simulink model "EV6_LUT_FourWheel_EV6Battery77p4kWh_PowerCorrected"  (R2024a)
settings: Solver=ode4  StartTime=0  StopTime=60  FixedStep=0.001  RelTol=1e-3
PreLoadFcn:
  | VSS_BICYCLE=Simulink.Variant('Dual=0');
  | VSS_DUAL=Simulink.Variant('Dual=1');
  | Dual=1;
  | load('DriveCycle2.mat')
PostLoadFcn:
  | if any(exist('dsrtsu_mdlpostloadfcn', 'file') ~= 0), dsrtsu_mdlpostloadfcn('Execute', bdroot); end
InitFcn:
  | , if any(exist('rtifpga_mdlclblib', 'file') ~= 0), rtifpga_mdlclblib('Init', bdroot); end,
  | , if any(exist('dsmpb_private', 'file') ~= 0), dsmpb_private('dsmpb_mdlclblib', 'Init', bdroot); end,
  | load('DriveCycle2.mat')
model workspace (MAT data in the model file):
  DiffRatio = 10.65
  EV6_2023_BattBranchCapacity_Ah = 55.5236728838
  EV6_2023_BattEnergy_kWh = 77.4
  EV6_2023_BattNominalVoltage_V = 697
  EV6_2023_BattNumCellsParallel = 2
  EV6_2023_BattNumCellsSeries = 192
  EV6_2023_BattOpenVoltCapBpts = [0 0.1 0.2 0.3 0.4 0.5 0.6 0.7 0.8 0.9 1]
  EV6_2023_BattOpenVoltTbl = [2.96762142548 3.40364281191 3.47417488548 3.54470541822 3.61523441014 3.68576186124 3.75628777151 3.82681214095 3.94527005036 4.07101207308 4.2120755254]
  EV6_2023_BattPackCapacity_Ah = 111.047345768
  EV6_2023_BattResistSocBpts = [0 0.2 0.4 0.6 0.8 1]
  EV6_2023_BattResistTbl = [0.0163620057716 0.0118174152018 0.00807187352333 0.00375663957972 0.00266904525531 0.00103635901355 0.0019014404175 0.0172368903217 0.0121226074867 0.00758541551769 0.00474065349228 0.00337561163613 ... (42 elements, 7x6)]
  EV6_2023_BattResistTempBpts = [243.1 253.1 263.1 273.1 283.1 298.1 313.1]
  EV6_2023_InitialPackOCV_V = 726.471714233
  EV6_2023_InitialSOC = 0.638878863672
  EV6_BattCellCapacity_Ah = 60.3
  EV6_BattInitialSOC = 0.638878863672
  EV6_BattOCV_Cell_V = [2.96762142548 3.40364281191 3.47417488548 3.54470541822 3.61523441014 3.68576186124 3.75628777151 3.82681214095 3.94527005036 4.07101207308 4.2120755254]
  EV6_BattOCV_SOC = [0 0.1 0.2 0.3 0.4 0.5 0.6 0.7 0.8 0.9 1]
  EV6_BattPackCapacity_Ah = 120.6
  EV6_BattParallelCells = 2
  EV6_BattResistanceSOC = [0 0.2 0.4 0.6 0.8 1]
  EV6_BattResistanceTable_Ohm = [0.0163620057716 0.0118174152018 0.00807187352333 0.00375663957972 0.00266904525531 0.00103635901355 0.0019014404175 0.0172368903217 0.0121226074867 0.00758541551769 0.00474065349228 0.00337561163613 ... (42 elements, 7x6)]
  EV6_BattResistanceTemp_K = [243.1 253.1 263.1 273.1 283.1 298.1 313.1]
  EV6_BattSeriesCells = 192
  EV6_FinalDriveRatio = 10.65
  EV6_TargetPackResistance_Ohm = 0.132763804608
  Gas = 0.383333333333
undefined symbols (not defined in the file): accel_bp_mps2, AccelCmd, ActTqLF_Nm_, ActTqLR_Nm_, ActTqRF_Nm_, ActTqRR_Nm_, BattChargeLimitMaxPwr, BattChargeLimitSocBpts, BattChargeLimitTbl, BattDischargeLimitSocBpts, BattDischargeLimitTbl, BattDischargeMaxPwr, BrakeMaxPrs, BrakeMaxTrq, ChassisDistCg2FrontAxle, ChassisDistCg2RearAxle, ChassisVehMass, CltchCmd, CoastDown, DecelCmd, DiscIntNeverNeededParam, EnvGravCnst, EnvPrs, EnvTemp, EV6_RegenTorqueGain, EV6_TractionTorqueGain, front_share_regen_3d, front_share_traction_3d, FuelSpecificGrav, GearCmd, h, InitStates, lgSw, limitedMCT, MCT, MtrEffSpdBpts, MtrEffTbl, MtrEffTrqBpts, MtrPwrMax, MtrTrqMax, out_1, pMCT, RealSimPara, Ref_speed, Ref_time, regen_torque_bp_Nm, speed_bp_kph, SteeringCmd, SupvsryCtrlRegenBrkCutOffTbl, SupvsryCtrlRegenSpdBpts, TestScnrioCycleNum, traction_torque_bp_Nm, US06, VEH
libraries: VSIGenLib x65, simulink x54, etargetslib x38, dsmpblib x24, vehdynlibtire x12, autolibshared x11, vehdynlibsuspension x7, vehdynlibtirecommon x7, autolibpowerinfoutils x6, autolibutils x5, autolibsharedcoupling x4, autolibmappedmotor x4
(part 2 of 19)

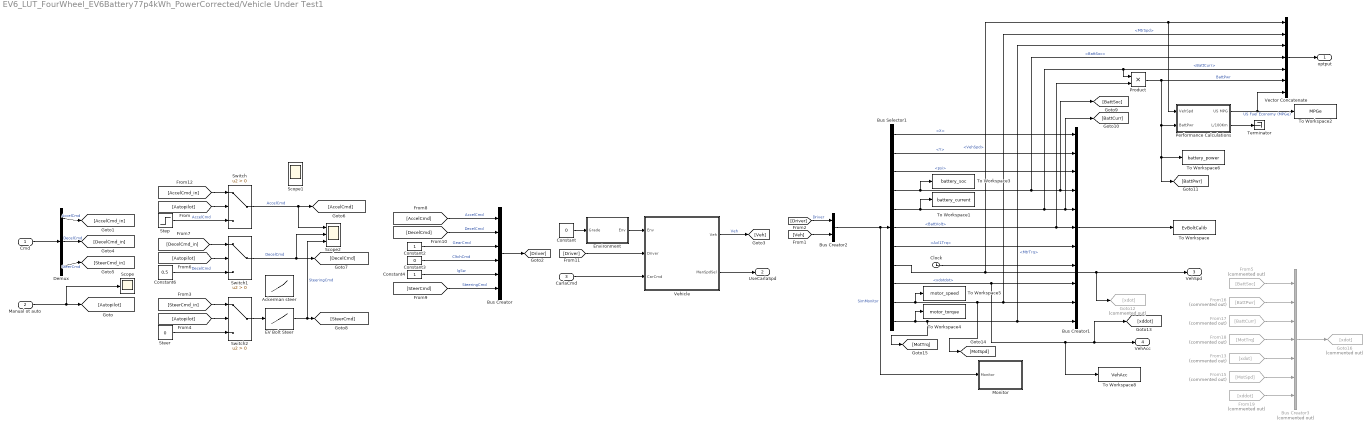
== system EV6_LUT_FourWheel_EV6Battery77p4kWh_PowerCorrected/Vehicle Under Test1 ==
  Cmd : Inport
  Manual ot auto : Inport  Port=2
  CarlaCmd : Inport  Port=3
  Ackerman steer : Lookup_n-D  NumberOfTableDimensions=1  BreakpointsForDimension1="[-0.446316297916244\t-0.442150786830951\t-0.437977161945005\t-0.433795286969319\t-0.429605025209166\t-0.425406239561593\t-0.421198792513030\t-0.416982546137136\t-0.412757362092861\t-0.408523101622746\t-0.404279625551461\t-0.400026794284603\t-0.395764467807732\t-0.391492505685692\t-0.387210767062193\t-0.382919110659678\t-0.378617394779480\t-0.374305477302279\t-0.369983215688866\t-0.365650466981227\t-0.361307087803951\t-0.356952934365975\t-0.352587862462675\t-0.348211727478321\t-0.343824384388886\t-0.339425687765245\t-0.335015491776758\t-0.330593650195247\t-0.326160016399396\t-0.321714443379563\t-0.317256783743034\t-0.312786889719717\t-0.308304613168298\t-0.303809805582871\t-0.299302318100048\t-0.294782001506567\t-0.290248706247410\t-0.285702282434450\t-0.281142579855627\t-0.276569447984685\t-0.271982735991464\t-0.267382292752788\t-0.262767966863931\t-0.258139606650706\t-0.253497060182174\t-0.248840175283994\t-0.244168799552432\t-0.239482780369037\t-0.234781964916014\t-0.230066200192295\t-0.225335333030331\t-0.220589210113630\t-0.215827677995039\t-0.211050583115807\t-0.206257771825433\t-0.201449090402323\t-0.196624385075265\t-0.191783502045761\t-0.186926287511198\t-0.182052587688919\t-0.177162248841170\t-0.172255117300976\t-0.167331039498945\t-0.162389861991014\t-0.157431431487183\t-0.152455594881217\t-0.147462199281363\t-0.142451092042095\t-0.137422120796894\t-0.132375133492088\t-0.127309978421782\t-0.122226504263869\t-0.117124560117169\t-0.112003995539695\t-0.106864660588066\t-0.101706405858090\t-0.0965290825265349\t-0.0913325423940914\t-0.0861166379295599\t-0.0808812223152671\t-0.0756261494937309\t-0.0703512742155897\t-0.0650564520888085\t-0.0597415396291770\t-0.0544063943121130\t-0.0490508746257825\t-0.0436748401255510\t-0.0382781514897739\t-0.0328606705769398\t-0.0274222604841732\t-0.0219627856071077\t-0.0164821117011354\t-0.0109801059440403\t-0.00545663700002112\t0\t0.00547767577609933\t0.0110656090794470\t0.0166755107772618\t0.0223075038233658\t0.0279617092740365\t0.0336382462142580\t0.0393372316825870\t0.0450587805946413\t0.0508030056652199\t0.0565700173290652\t0.0623599236602815\t0.0681728302904245\t0.0740088403252790\t0.0798680542603446\t0.0857505698950509\t0.0916564822457268\t0.0975858834573503\t0.103538862714108\t0.109515506148794\t0.115515896751090\t0.121540114274751\t0.127588235143750\t0.133660332357415\t0.139756475394610\t0.145876730117007\t0.152021158671496\t0.158189819391799\t0.164382766699339\t0.170600051003425\t0.176841718600822\t0.183107811574771\t0.189398367693541\t0.195713420308563\t0.202052998252265\t0.208417125735647\t0.214805822245717\t0.221219102442855\t0.227656976058216\t0.234119447791246\t0.240606517207442\t0.247118178636427\t0.253654421070478\t0.260215228063589\t0.266800577631217\t0.273410442150791\t0.280044788263140\t0.286703576774936\t0.293386762562311\t0.300094294475738\t0.306826115246357\t0.313582161393837\t0.320362363135953\t0.327166644299990\t0.333994922236136\t0.340847107733006\t0.347723104935443\t0.354622811264752\t0.361546117341510\t0.368492906911125\t0.375463056772267\t0.382456436708368\t0.389472909422305\t0.396512330474460\t0.403574548224288\t0.410659403775562\t0.417766730925451\t0.424896356117582\t0.432048098399246\t0.439221769382891\t0.446417173212069\t0.453634106531970\t0.460872358464695\t0.468131710589418\t0.475411936927561\t0.482712803933137\t0.490034070488372\t0.497375487904758\t0.504736799929627\t0.512117742758400\t0.519518045052588\t0.526937427963674\t0.534375605162959\t0.541832282877473\t0.549307159932028\t0.556799927797496\t0.564310270645373\t0.571837865408689\t0.579382381849329\t0.586943482631776\t0.594520823403350\t0.602114052880920\t0.609722812944144\t0.617346738735206\t0.624985458765058]"  Table="[-9.40000000000000\t-9.30000000000000\t-9.20000000000000\t-9.10000000000000\t-9\t-8.90000000000000\t-8.80000000000000\t-8.70000000000000\t-8.60000000000000\t-8.50000000000000\t-8.40000000000000\t-8.30000000000000\t-8.20000000000000\t-8.10000000000000\t-8\t-7.90000000000000\t-7.80000000000000\t-7.70000000000000\t-7.60000000000000\t-7.50000000000000\t-7.40000000000000\t-7.30000000000000\t-7.20000000000000\t-7.10000000000000\t-7\t-6.90000000000000\t-6.80000000000000\t-6.70000000000000\t-6.60000000000000\t-6.50000000000000\t-6.40000000000000\t-6.30000000000000\t-6.20000000000000\t-6.10000000000000\t-6\t-5.90000000000000\t-5.80000000000000\t-5.70000000000000\t-5.60000000000000\t-5.50000000000000\t-5.40000000000000\t-5.30000000000000\t-5.20000000000000\t-5.10000000000000\t-5\t-4.90000000000000\t-4.80000000000000\t-4.70000000000000\t-4.60000000000000\t-4.50000000000000\t-4.40000000000000\t-4.30000000000000\t-4.20000000000000\t-4.10000000000000\t-4\t-3.90000000000000\t-3.80000000000000\t-3.70000000000000\t-3.60000000000000\t-3.50000000000000\t-3.40000000000000\t-3.30000000000000\t-3.20000000000000\t-3.10000000000000\t-3\t-2.90000000000000\t-2.80000000000000\t-2.70000000000000\t-2.60000000000000\t-2.50000000000000\t-2.40000000000000\t-2.30000000000000\t-2.20000000000000\t-2.10000000000000\t-2\t-1.90000000000000\t-1.80000000000000\t-1.70000000000000\t-1.60000000000000\t-1.50000000000000\t-1.40000000000000\t-1.30000000000000\t-1.20000000000000\t-1.10000000000000\t-1\t-0.900000000000000\t-0.800000000000000\t-0.700000000000000\t-0.600000000000000\t-0.500000000000000\t-0.400000000000000\t-0.300000000000000\t-0.200000000000000\t-0.100000000000000\t0\t0.100000000000000\t0.200000000000000\t0.300000000000000\t0.400000000000000\t0.500000000000000\t0.600000000000000\t0.700000000000000\t0.800000000000000\t0.900000000000000\t1\t1.10000000000000\t1.20000000000000\t1.30000000000000\t1.40000000000000\t1.50000000000000\t1.60000000000000\t1.70000000000000\t1.80000000000000\t1.90000000000000\t2\t2.10000000000000\t2.20000000000000\t2.30000000000000\t2.40000000000000\t2.50000000000000\t2.60000000000000\t2.70000000000000\t2.80000000000000\t2.90000000000000\t3\t3.10000000000000\t3.20000000000000\t3.30000000000000\t3.40000000000000\t3.50000000000000\t3.60000000000000\t3.70000000000000\t3.80000000000000\t3.90000000000000\t4\t4.10000000000000\t4.20000000000000\t4.30000000000000\t4.40000000000000\t4.50000000000000\t4.60000000000000\t4.70000000000000\t4.80000000000000\t4.90000000000000\t5\t5.10000000000000\t5.20000000000000\t5.30000000000000\t5.40000000000000\t5.50000000000000\t5.60000000000000\t5.70000000000000\t5.80000000000000\t5.90000000000000\t6\t6.10000000000000\t6.20000000000000\t6.30000000000000\t6.40000000000000\t6.50000000000000\t6.60000000000000\t6.70000000000000\t6.80000000000000\t6.90000000000000\t7\t7.10000000000000\t7.20000000000000\t7.30000000000000\t7.40000000000000\t7.50000000000000\t7.60000000000000\t7.70000000000000\t7.80000000000000\t7.90000000000000\t8\t8.10000000000000\t8.20000000000000\t8.30000000000000\t8.40000000000000\t8.50000000000000\t8.60000000000000\t8.70000000000000\t8.80000000000000\t8.90000000000000\t9\t9.10000000000000\t9.20000000000000\t9.30000000000000\t9.40000000000000]"  InternalRulePriority=Speed  RndMeth=Simplest
  Bus Creator : BusCreator  Inputs=AccelCmd,DecelCmd,GearCmd,CltchCmd,lgSw,SteeringCmd
  Bus Creator1 : BusCreator  Inputs=11
  Bus Creator2 : BusCreator  Inputs=2
  Bus Creator3 : BusCreator  Commented=on  Inputs=7
  Bus Selector1 : BusSelector  OutputSignals=Veh.Chassis.X,Veh.Chassis.Y,Veh.Chassis.psi,Veh.Batt.BattSoc,Veh.Batt.BattCurr,Veh.Batt.BattVolt,Veh.Diff.Axl1.Axl1Trq,Veh.Chassis.VehSpd,Veh.Chassis.xdotdot,Veh.Mtr.MtrSpd,Veh.Mtr.MtrTrq
  Clock : Clock
  Constant : Constant  Value=0
  Constant2 : Constant
  Constant3 : Constant  Value=0
  Constant4 : Constant
  Constant6 : Constant  Value=0.5  SampleTime=-1
  Demux : Demux  Outputs=3
  EV Bolt Steer : Lookup_n-D  NumberOfTableDimensions=1  BreakpointsForDimension1="[-0.541571931581492\t-0.535619550629112\t-0.529667169676731\t-0.523714788724350\t-0.517762407771969\t-0.511810026819588\t-0.505857645867207\t-0.499905264914826\t-0.493952883962445\t-0.488000503010064\t-0.482048122057683\t-0.476095741105302\t-0.470143360152921\t-0.464190979200541\t-0.458238598248160\t-0.452286217295779\t-0.446333836343398\t-0.440381455391017\t-0.434429074438636\t-0.428476693486255\t-0.422524312533874\t-0.416571931581493\t-0.410619550629112\t-0.404667169676731\t-0.398714788724350\t-0.392762407771969\t-0.386810026819588\t-0.380857645867207\t-0.374905264914826\t-0.368952883962445\t-0.363000503010064\t-0.357048122057683\t-0.351095741105302\t-0.345143360152921\t-0.339190979200541\t-0.333238598248160\t-0.327286217295779\t-0.321333836343398\t-0.315381455391017\t-0.309429074438636\t-0.303476693486255\t-0.297524312533874\t-0.291571931581493\t-0.285619550629112\t-0.279667169676731\t-0.273714788724350\t-0.267762407771969\t-0.261810026819588\t-0.255857645867207\t-0.249905264914826\t-0.243952883962445\t-0.238000503010065\t-0.232048122057684\t-0.226095741105303\t-0.220143360152922\t-0.214190979200541\t-0.208238598248160\t-0.202286217295779\t-0.196333836343398\t-0.190381455391017\t-0.184429074438636\t-0.178476693486255\t-0.172524312533874\t-0.166571931581493\t-0.160619550629112\t-0.154667169676731\t-0.148714788724350\t-0.142762407771969\t-0.136810026819588\t-0.130857645867207\t-0.124905264914826\t-0.118952883962445\t-0.113000503010064\t-0.107048122057683\t-0.101095741105303\t-0.0951433601529216\t-0.0891909792005406\t-0.0832385982481596\t-0.0772862172957787\t-0.0713338363433977\t-0.0653814553910168\t-0.0594290744386358\t-0.0534766934862548\t-0.0475243125338739\t-0.0415719315814929\t-0.0356195506291120\t-0.0296671696767310\t-0.0237147887243500\t-0.0177624077719691\t-0.0118100268195881\t-0.00585764586720720\t0\t0.00585764586720720\t0.0118100268195881\t0.0177624077719691\t0.0237147887243500\t0.0296671696767310\t0.0356195506291120\t0.0415719315814929\t0.0475243125338739\t0.0534766934862548\t0.0594290744386358\t0.0653814553910168\t0.0713338363433977\t0.0772862172957787\t0.0832385982481596\t0.0891909792005406\t0.0951433601529216\t0.101095741105303\t0.107048122057683\t0.113000503010064\t0.118952883962445\t0.124905264914826\t0.130857645867207\t0.136810026819588\t0.142762407771969\t0.148714788724350\t0.154667169676731\t0.160619550629112\t0.166571931581493\t0.172524312533874\t0.178476693486255\t0.184429074438636\t0.190381455391017\t0.196333836343398\t0.202286217295779\t0.208238598248160\t0.214190979200541\t0.220143360152922\t0.226095741105303\t0.232048122057684\t0.238000503010065\t0.243952883962445\t0.249905264914826\t0.255857645867207\t0.261810026819588\t0.267762407771969\t0.273714788724350\t0.279667169676731\t0.285619550629112\t0.291571931581493\t0.297524312533874\t0.303476693486255\t0.309429074438636\t0.315381455391017\t0.321333836343398\t0.327286217295779\t0.333238598248160\t0.339190979200541\t0.345143360152921\t0.351095741105302\t0.357048122057683\t0.363000503010064\t0.368952883962445\t0.374905264914826\t0.380857645867207\t0.386810026819588\t0.392762407771969\t0.398714788724350\t0.404667169676731\t0.410619550629112\t0.416571931581493\t0.422524312533874\t0.428476693486255\t0.434429074438636\t0.440381455391017\t0.446333836343398\t0.452286217295779\t0.458238598248160\t0.464190979200541\t0.470143360152921\t0.476095741105302\t0.482048122057683\t0.488000503010064\t0.493952883962445\t0.499905264914826\t0.505857645867207\t0.511810026819588\t0.517762407771969\t0.523714788724350\t0.529667169676731\t0.535619550629112\t0.541571931581492]"  Table="[-9.10000000000000\t-9\t-8.90000000000000\t-8.80000000000000\t-8.70000000000000\t-8.60000000000000\t-8.50000000000000\t-8.40000000000000\t-8.30000000000000\t-8.20000000000000\t-8.10000000000000\t-8\t-7.90000000000000\t-7.80000000000000\t-7.70000000000000\t-7.60000000000000\t-7.50000000000000\t-7.40000000000000\t-7.30000000000000\t-7.20000000000000\t-7.10000000000000\t-7\t-6.90000000000000\t-6.80000000000000\t-6.70000000000000\t-6.60000000000000\t-6.50000000000000\t-6.40000000000000\t-6.30000000000000\t-6.20000000000000\t-6.10000000000000\t-6\t-5.90000000000000\t-5.80000000000000\t-5.70000000000000\t-5.60000000000000\t-5.50000000000000\t-5.40000000000000\t-5.30000000000000\t-5.20000000000000\t-5.10000000000000\t-5\t-4.90000000000000\t-4.80000000000000\t-4.70000000000000\t-4.60000000000000\t-4.50000000000000\t-4.40000000000000\t-4.30000000000000\t-4.20000000000000\t-4.10000000000000\t-4\t-3.90000000000000\t-3.80000000000000\t-3.70000000000000\t-3.60000000000000\t-3.50000000000000\t-3.40000000000000\t-3.30000000000000\t-3.20000000000000\t-3.10000000000000\t-3\t-2.90000000000000\t-2.80000000000000\t-2.70000000000000\t-2.60000000000000\t-2.50000000000000\t-2.40000000000000\t-2.30000000000000\t-2.20000000000000\t-2.10000000000000\t-2\t-1.90000000000000\t-1.80000000000000\t-1.70000000000000\t-1.60000000000000\t-1.50000000000000\t-1.40000000000000\t-1.30000000000000\t-1.20000000000000\t-1.10000000000000\t-1\t-0.900000000000000\t-0.800000000000000\t-0.700000000000000\t-0.600000000000000\t-0.500000000000000\t-0.400000000000000\t-0.300000000000000\t-0.200000000000000\t-0.100000000000000\t0\t0.100000000000000\t0.200000000000000\t0.300000000000000\t0.400000000000000\t0.500000000000000\t0.600000000000000\t0.700000000000000\t0.800000000000000\t0.900000000000000\t1\t1.10000000000000\t1.20000000000000\t1.30000000000000\t1.40000000000000\t1.50000000000000\t1.60000000000000\t1.70000000000000\t1.80000000000000\t1.90000000000000\t2\t2.10000000000000\t2.20000000000000\t2.30000000000000\t2.40000000000000\t2.50000000000000\t2.60000000000000\t2.70000000000000\t2.80000000000000\t2.90000000000000\t3\t3.10000000000000\t3.20000000000000\t3.30000000000000\t3.40000000000000\t3.50000000000000\t3.60000000000000\t3.70000000000000\t3.80000000000000\t3.90000000000000\t4\t4.10000000000000\t4.20000000000000\t4.30000000000000\t4.40000000000000\t4.50000000000000\t4.60000000000000\t4.70000000000000\t4.80000000000000\t4.90000000000000\t5\t5.10000000000000\t5.20000000000000\t5.30000000000000\t5.40000000000000\t5.50000000000000\t5.60000000000000\t5.70000000000000\t5.80000000000000\t5.90000000000000\t6\t6.10000000000000\t6.20000000000000\t6.30000000000000\t6.40000000000000\t6.50000000000000\t6.60000000000000\t6.70000000000000\t6.80000000000000\t6.90000000000000\t7\t7.10000000000000\t7.20000000000000\t7.30000000000000\t7.40000000000000\t7.50000000000000\t7.60000000000000\t7.70000000000000\t7.80000000000000\t7.90000000000000\t8\t8.10000000000000\t8.20000000000000\t8.30000000000000\t8.40000000000000\t8.50000000000000\t8.60000000000000\t8.70000000000000\t8.80000000000000\t8.90000000000000\t9\t9.10000000000000]"  InternalRulePriority=Speed  RndMeth=Simplest
  Environment : Subsystem
  From13 : From  Commented=on  GotoTag=xdot
  From15 : From  Commented=on  GotoTag=MotSpd
  From16 : From  Commented=on  GotoTag=BattPwr
  From17 : From  Commented=on  GotoTag=BattCurr
  From18 : From  Commented=on  GotoTag=MotTrq
  From19 : From  Commented=on  GotoTag=xddot
  From5 : From  Commented=on  GotoTag=BattSoc
  Goto12 : Goto  Commented=on  GotoTag=xdot
  Goto16 : Goto  Commented=on  GotoTag=xdot
  Monitor : Subsystem
  Performance Calculations : Subsystem
  Product : Product
  Scope : Scope
  Scope1 : Scope  NumInputPorts=3
  Scope2 : Scope  NumInputPorts=3
  Steer : Constant  Value=0
  Step : Step  Time=5  After=0
  Switch : Switch  Criteria=u2 > Threshold  SaturateOnIntegerOverflow=off  InputSameDT=off
  Switch1 : Switch  Criteria=u2 > Threshold  SaturateOnIntegerOverflow=off  InputSameDT=off
  Switch2 : Switch  Criteria=u2 > Threshold  SaturateOnIntegerOverflow=off  InputSameDT=off
  Terminator : Terminator
  To Workspace : ToWorkspace  VariableName=EvBoltCalib  SaveFormat=Structure With Time  SampleTime=-1
  To Workspace1 : ToWorkspace  VariableName=battery_current  SaveFormat=Timeseries  SampleTime=0.1
  To Workspace2 : ToWorkspace  VariableName=MPGe  SaveFormat=Timeseries  SampleTime=0.1
  To Workspace3 : ToWorkspace  VariableName=battery_soc  SaveFormat=Timeseries  SampleTime=0.1
  To Workspace4 : ToWorkspace  VariableName=motor_torque  SaveFormat=Timeseries  SampleTime=0.1
  To Workspace5 : ToWorkspace  VariableName=motor_speed  SaveFormat=Timeseries  SampleTime=0.1
  To Workspace6 : ToWorkspace  VariableName=battery_power  SaveFormat=Timeseries  SampleTime=0.1
  To Workspace8 : ToWorkspace  VariableName=VehAcc  SaveFormat=Timeseries  SampleTime=0.1
  Vector Concatenate : Concatenate  NumInputs=7
  Vehicle : Subsystem
  optput : Outport
  UseCarlaSpd : Outport  Port=2
  VehSpd : Outport  Port=3
  VehAcc : Outport  Port=4
  wires:
  Performance Calculations/2(L/100Km) -> Terminator/1
  Performance Calculations/1(US MPG) -> Vector Concatenate/7, To Workspace2/1  "US Fuel Economy (MPGe)"
  Product/1 -> Vector Concatenate/6, Performance Calculations/2(BattPwr), [BattPwr], To Workspace6/1  "BattPwr"
  Bus Selector1/11 -> [MotTrq], Vector Concatenate/3, Bus Creator1/11, To Workspace4/1  "<MtrTrq>"
  Bus Selector1/10 -> [MotSpd], Vector Concatenate/2, Bus Creator1/10, To Workspace5/1  "<MtrSpd>"
  [Driver] -> Vehicle/2(Driver)
  [DecelCmd] -> Bus Creator/2  "DecelCmd"
  EV Bolt Steer/1 -> [SteerCmd], Scope2/3  "SteeringCmd"
  [AccelCmd] -> Bus Creator/1  "AccelCmd"
  [DecelCmd_in] -> Switch1/1
  [Autopilot] -> Switch1/2
  [SteerCmd_in] -> Switch2/1
  [Autopilot] -> Switch2/2
  [AccelCmd_in] -> Switch/1
  Bus Selector1/9 -> To Workspace8/1, [xddot], VehAcc/1, Bus Creator1/9  "<xdotdot>"
  [Veh] -> Bus Creator2/2
  Vehicle/2(ManSpdSel) -> UseCarlaSpd/1
  CarlaCmd/1 -> Vehicle/3(CarCmd)
  Demux/3 -> [SteerCmd_in]  "SteerCmd"
  Steer/1 -> Switch2/3
  Demux/2 -> [DecelCmd_in]  "DecelCmd"
  Constant6/1 -> Switch1/3  "DecelCmd"
  Demux/1 -> [AccelCmd_in]  "AccelCmd"
  Step/1 -> Switch/3  "AccelCmd"
  [Autopilot] -> Switch/2
  Manual ot auto/1 -> [Autopilot], Scope/1
  Switch1/1 -> [DecelCmd], Scope2/2  "DecelCmd"
  Switch/1 -> [AccelCmd], Scope2/1  "AccelCmd"
  Switch2/1 -> EV Bolt Steer/1
  [SteerCmd] -> Bus Creator/6  "SteeringCmd"
  Bus Selector1/8 -> Vector Concatenate/1, Performance Calculations/1(VehSpd), Goto12/1, VehSpd/1  "<VehSpd>"
  Bus Selector1/7 -> Bus Creator1/7  "<Axl1Trq>"
  Bus Selector1/6 -> Bus Creator1/6, Product/2  "<BattVolt>"
  Bus Selector1/5 -> [BattCurr], Bus Creator1/5, Vector Concatenate/5, Product/1, To Workspace1/1  "<BattCurr>"
  Bus Selector1/4 -> Vector Concatenate/4, [BattSoc], Bus Creator1/4, To Workspace3/1  "<BattSoc>"
  Bus Selector1/3 -> Bus Creator1/3  "<psi>"
  Bus Selector1/2 -> Bus Creator1/2  "<Y>"
  Bus Selector1/1 -> Bus Creator1/1  "<X>"
  Clock/1 -> Bus Creator1/8
  Vector Concatenate/1 -> optput/1
  Constant2/1 -> Bus Creator/3  "GearCmd"
  Bus Creator1/1 -> To Workspace/1
  Constant4/1 -> Bus Creator/5  "lgSw"
  Constant/1 -> Environment/1(Grade)
  Environment/1(Env) -> Vehicle/1(Env)
  Vehicle/1(Veh) -> [Veh]  "Veh"
  Bus Creator/1 -> [Driver]
  Cmd/1 -> Demux/1
  Constant3/1 -> Bus Creator/4  "CltchCmd"
  [Driver] -> Bus Creator2/1  "Driver"
  Bus Creator2/1 -> Bus Selector1/1, Monitor/1(Monitor)  "SimMonitor"
  From5/1 -> Bus Creator3/1
  From16/1 -> Bus Creator3/2
  From17/1 -> Bus Creator3/3
  From18/1 -> Bus Creator3/4
  From13/1 -> Bus Creator3/5
  From15/1 -> Bus Creator3/6
  From19/1 -> Bus Creator3/7
  Bus Creator3/1 -> Goto16/1

== system EV6_LUT_FourWheel_EV6Battery77p4kWh_PowerCorrected/RealSim1/FromRealSim ==
  note: RealSimDepack
      | INPUTS
      | 0: uint8 ByteData array, this is message received from TrafficLayer
      | 1: nByte received
      |
      | The OUTPUTS can be customized based on the needs. Check SourceCode of this block for details.
  note: RealSimSocket
      | PARAMETERS:
      | 0: ip address of the RealSim TrafficLayer
      | 1: port to RealSim TrafficLayer
      | 2: enable log or not, disable for performance
      | INPUT:
      | 0: simulation time
      | 1: dt, frequency to receive and send to Traffic Simulator, has to be 0.1 for now, DO NOT change
      | 2: enable connection, 1: enable, 0: close. NOT currently used.
      | 3: ByteData to send
      | 4: nMsgSize
      |
      | OUTPUT:
      | 0: uint8 ByteData array
      | 1: nByte received
      | 2: connection flag, 1: connected to TrafficSimulator, 0: not connected
  tSimu : Inport
  dt : Inport  Port=2
  enableConnection : Inport  Port=3
  byteDataOut : Inport  Port=4
  nMsgSizeOut : Inport  Port=5
  Data Type Conversion1 : DataTypeConversion  OutDataTypeStr=uint8  SaturateOnIntegerOverflow=off  RndMeth=Floor
  Data Type Conversion2 : DataTypeConversion  OutDataTypeStr=boolean  SaturateOnIntegerOverflow=off  RndMeth=Floor
  Data Type Conversion3 : DataTypeConversion  OutDataTypeStr=double  SaturateOnIntegerOverflow=off  RndMeth=Floor
  Display8 : Display
  MATLAB System : MATLABSystem  System=RealSimDepack  OutputBusName=VehDataBus  VehicleMessageFieldDefInputVec=VehicleMessageFieldDefInputVec  SimulateUsing=Interpreted execution
      mask Type: RealSimDepack
      mask Display:
      | disp('RealSimDepack');
      | port_label('input',1,'ByteData');
      | port_label('input',2,'nByte');
      | port_label('input',3,'connectionState');
      | port_label('output',1,'simState');
      | port_label('output',2,'t');
      | port_label('output',3,'nVeh');
      | port_label('output',4,'VehDataBus');
      | port_label('output',5,'isVehicleInNetwork');
  S-Function : S-Function  FunctionName=RealSimSocket  Parameters=TrafficLayerIP, TrafficLayerPort, 1  SFunctionDeploymentMode=off  EnableBusSupport=off
  Signal Specification : SignalSpecification  Dimensions=[2048 1]
  simState : Outport
  t : Outport  Port=2
  nVeh : Outport  Port=3
  VehDataBus : Outport  Port=4
  isVehicleInNetwork : Outport  Port=5
  connectionState : Outport  Port=6
  wires:
  Data Type Conversion3/1 -> MATLAB System/3, [connectionState], connectionState/1
  enableConnection/1 -> Data Type Conversion2/1
  dt/1 -> S-Function/2
  tSimu/1 -> S-Function/1
  MATLAB System/5 -> isVehicleInNetwork/1
  MATLAB System/3 -> nVeh/1
  MATLAB System/1 -> simState/1
  MATLAB System/4 -> VehDataBus/1
  S-Function/1 -> Data Type Conversion1/1
  Data Type Conversion2/1 -> S-Function/3
  Signal Specification/1 -> S-Function/4
  S-Function/2 -> MATLAB System/2, Display8/1
  Data Type Conversion1/1 -> MATLAB System/1
  byteDataOut/1 -> Signal Specification/1
  MATLAB System/2 -> t/1
  S-Function/3 -> Data Type Conversion3/1
  nMsgSizeOut/1 -> S-Function/5

== system EV6_LUT_FourWheel_EV6Battery77p4kWh_PowerCorrected/RealSim1/SwitchVehicleSpeed ==
  speedIn : Inport
  initialSpeed : Inport  Port=2
  Clock : Clock
  Switch : Switch  Criteria=u2 > Threshold  Threshold=RealSimPara.warmupTime  SaturateOnIntegerOverflow=off  InputSameDT=off
  speedCmd : Outport
  wires:
  initialSpeed/1 -> Switch/3
  Clock/1 -> Switch/2
  speedIn/1 -> Switch/1
  Switch/1 -> speedCmd/1

== system EV6_LUT_FourWheel_EV6Battery77p4kWh_PowerCorrected/RealSim1/ToRealSim ==
  note: RealSimPack
      | INPUTS
      | 1. simState: always set to 1. NOT actively used.
      | 2. t: simulation time
      | 3. speedDesired: desired speed in m/s, For Toyota, leave as 0.
      | 4. accelerationDesired: desired acceleration in m/s^2
      | 5. id: string of the vehicle id, will be received from RealSimDepack and as one of its output.
      | 6. idLength: length of the vehicle id string, will be received from RealSimDepack and as one of its outputs
      | 7: activeLaneChange: activeLaneChange command, 0: no lane change, +1: change to left lane, -1: change to right lane. NOTE: need to reset activeLaneChange to 0 after lane change finishes, otherwise vehicle will keep making lane change. Will receive 0 activeLaneChangeFdbk from RealSimDepack when lane change finishes.
      |
      | NOTE 1: Currently, only speedDesired and/or accelerationDesired can be sent to VISSIM/SUMO. The data format receive and send are the same so other mesage fields of the send data are irrelevant and can be set to empty or zero.
      |
      | NOTE 2: if select both speedDesired and accelerationDesired
      | in config.yaml, then only accelerationDesired will be used
      | to control vehicles in TrafficSimulator. if only one of
      | speedDesired and accelerationDesired selected in
      | config.yaml, then the one selected will be used for
      | control, the other input can be leave as 0.
      |
      | NOTE 3: for VISSIM, speedDesired or accelerationDesired will be the control command 0.2 seconds in the future.
      |
      | OUTPUTS
      | 1.ByteData: bytes vector that will be sent to TrafficSimualtor
      | 2.nMsgSize: size of bytes to be sent
  In1 : Inport
  In2 : Inport  Port=2
  In3 : Inport  Port=3
  accelerationDesired : Inport  Port=4
  MATLAB System1 : MATLABSystem  System=RealSimPack  VehicleMessageFieldDefInputVec=VehicleMessageFieldDefInputVec  SimulateUsing=Code generation
      mask Type: RealSimPack
      mask Display:
      | disp('RealSimPack');
      | port_label('input',1,'simState');
      | port_label('input',2,'t');
      | port_label('input',3,'VehDataBus');
      | port_label('output',1,'ByteData');
      | port_label('output',2,'nMsgSize');
  RealSim CreatBus : Subsystem
  activeLaneChange : Constant  Value=0
  rgba : Constant  Value=[255,0,0,255]
  simState : Constant
  ByteSend : Outport
  nMsgSend : Outport  Port=2
  wires:
  In2/1 -> RealSim CreatBus/1(In)
  MATLAB System1/1 -> ByteSend/1  "ByteSend"
  activeLaneChange/1 -> RealSim CreatBus/5(activeLaneChange)
  RealSim CreatBus/1(Out) -> MATLAB System1/3
  accelerationDesired/1 -> RealSim CreatBus/4(accelerationDesired)
  simState/1 -> MATLAB System1/1
  In1/1 -> MATLAB System1/2
  In3/1 -> RealSim CreatBus/2(speedDesired)
  MATLAB System1/2 -> nMsgSend/1  "nMsgSend"
  rgba/1 -> RealSim CreatBus/3(color)

== system EV6_LUT_FourWheel_EV6Battery77p4kWh_PowerCorrected/RealSim2/FromRealSim ==
  note: RealSimDepack
      | INPUTS
      | 0: uint8 ByteData array, this is message received from TrafficLayer
      | 1: nByte received
      |
      | The OUTPUTS can be customized based on the needs. Check SourceCode of this block for details.
  note: RealSimSocket
      | PARAMETERS:
      | 0: ip address of the RealSim TrafficLayer
      | 1: port to RealSim TrafficLayer
      | 2: enable log or not, disable for performance
      | INPUT:
      | 0: simulation time
      | 1: dt, frequency to receive and send to Traffic Simulator, has to be 0.1 for now, DO NOT change
      | 2: enable connection, 1: enable, 0: close. NOT currently used.
      | 3: ByteData to send
      | 4: nMsgSize
      |
      | OUTPUT:
      | 0: uint8 ByteData array
      | 1: nByte received
      | 2: connection flag, 1: connected to TrafficSimulator, 0: not connected
  tSimu : Inport
  dt : Inport  Port=2
  enableConnection : Inport  Port=3
  byteDataOut : Inport  Port=4
  nMsgSizeOut : Inport  Port=5
  Data Type Conversion1 : DataTypeConversion  OutDataTypeStr=uint8  SaturateOnIntegerOverflow=off  RndMeth=Floor
  Data Type Conversion2 : DataTypeConversion  OutDataTypeStr=boolean  SaturateOnIntegerOverflow=off  RndMeth=Floor
  Data Type Conversion3 : DataTypeConversion  OutDataTypeStr=double  SaturateOnIntegerOverflow=off  RndMeth=Floor
  Display8 : Display
  MATLAB System : MATLABSystem  System=RealSimDepack  OutputBusName=VehDataBus  VehicleMessageFieldDefInputVec=VehicleMessageFieldDefInputVec  SimulateUsing=Interpreted execution
      mask Type: RealSimDepack
      mask Display:
      | disp('RealSimDepack');
      | port_label('input',1,'ByteData');
      | port_label('input',2,'nByte');
      | port_label('input',3,'connectionState');
      | port_label('output',1,'simState');
      | port_label('output',2,'t');
      | port_label('output',3,'nVeh');
      | port_label('output',4,'VehDataBus');
      | port_label('output',5,'isVehicleInNetwork');
  S-Function : S-Function  FunctionName=RealSimSocket  Parameters=TrafficLayerIP, TrafficLayerPort, 1  SFunctionDeploymentMode=off  EnableBusSupport=off
  Signal Specification : SignalSpecification  Dimensions=[200 1]
  simState : Outport
  t : Outport  Port=2
  nVeh : Outport  Port=3
  VehDataBus : Outport  Port=4
  isVehicleInNetwork : Outport  Port=5
  connectionState : Outport  Port=6
  wires:
  Data Type Conversion3/1 -> [connectionState], MATLAB System/3
  enableConnection/1 -> Data Type Conversion2/1
  dt/1 -> S-Function/2
  tSimu/1 -> S-Function/1
  MATLAB System/5 -> isVehicleInNetwork/1
  MATLAB System/3 -> nVeh/1
  MATLAB System/1 -> simState/1
  MATLAB System/4 -> VehDataBus/1
  S-Function/1 -> Data Type Conversion1/1
  Data Type Conversion2/1 -> S-Function/3
  Signal Specification/1 -> S-Function/4
  S-Function/2 -> MATLAB System/2, Display8/1
  Data Type Conversion1/1 -> MATLAB System/1
  byteDataOut/1 -> Signal Specification/1
  MATLAB System/2 -> t/1
  S-Function/3 -> Data Type Conversion3/1
  nMsgSizeOut/1 -> S-Function/5
  [connectionState] -> connectionState/1

== system EV6_LUT_FourWheel_EV6Battery77p4kWh_PowerCorrected/RealSim2/SwitchVehicleSpeed ==
  speedIn : Inport
  initialSpeed : Inport  Port=2
  Clock : Clock
  Switch : Switch  Criteria=u2 > Threshold  Threshold=RealSimPara.warmupTime  SaturateOnIntegerOverflow=off  InputSameDT=off
  speedCmd : Outport
  wires:
  initialSpeed/1 -> Switch/3
  Clock/1 -> Switch/2
  speedIn/1 -> Switch/1
  Switch/1 -> speedCmd/1

== system EV6_LUT_FourWheel_EV6Battery77p4kWh_PowerCorrected/RealSim2/ToRealSim ==
  note: RealSimPack
      | INPUTS
      | 1. simState: always set to 1. NOT actively used.
      | 2. t: simulation time
      | 3. speedDesired: desired speed in m/s, For Toyota, leave as 0.
      | 4. accelerationDesired: desired acceleration in m/s^2
      | 5. id: string of the vehicle id, will be received from RealSimDepack and as one of its output.
      | 6. idLength: length of the vehicle id string, will be received from RealSimDepack and as one of its outputs
      | 7: activeLaneChange: activeLaneChange command, 0: no lane change, +1: change to left lane, -1: change to right lane. NOTE: need to reset activeLaneChange to 0 after lane change finishes, otherwise vehicle will keep making lane change. Will receive 0 activeLaneChangeFdbk from RealSimDepack when lane change finishes.
      |
      | NOTE 1: Currently, only speedDesired and/or accelerationDesired can be sent to VISSIM/SUMO. The data format receive and send are the same so other mesage fields of the send data are irrelevant and can be set to empty or zero.
      |
      | NOTE 2: if select both speedDesired and accelerationDesired
      | in config.yaml, then only accelerationDesired will be used
      | to control vehicles in TrafficSimulator. if only one of
      | speedDesired and accelerationDesired selected in
      | config.yaml, then the one selected will be used for
      | control, the other input can be leave as 0.
      |
      | NOTE 3: for VISSIM, speedDesired or accelerationDesired will be the control command 0.2 seconds in the future.
      |
      | OUTPUTS
      | 1.ByteData: bytes vector that will be sent to TrafficSimualtor
      | 2.nMsgSize: size of bytes to be sent
  tIn : Inport
  VehDataBusIn : Inport  Port=2
  speedActual : Inport  Port=3
  accelerationDesired : Inport  Port=4
  MATLAB System1 : MATLABSystem  System=RealSimPack  VehicleMessageFieldDefInputVec=VehicleMessageFieldDefInputVec  SimulateUsing=Code generation
      mask Type: RealSimPack
      mask Display:
      | disp('RealSimPack');
      | port_label('input',1,'simState');
      | port_label('input',2,'t');
      | port_label('input',3,'VehDataBus');
      | port_label('output',1,'ByteData');
      | port_label('output',2,'nMsgSize');
  RealSim CreatBus : Subsystem
  activeLaneChange : Constant  Value=0
  rgba : Constant  Value=[255,0,0,255]
  simState : Constant
  ByteSend : Outport
  nMsgSend : Outport  Port=2
  wires:
  VehDataBusIn/1 -> RealSim CreatBus/1(In)
  MATLAB System1/1 -> ByteSend/1  "ByteSend"
  activeLaneChange/1 -> RealSim CreatBus/5(activeLaneChange)
  RealSim CreatBus/1(Out) -> MATLAB System1/3
  accelerationDesired/1 -> RealSim CreatBus/4(accelerationDesired)
  simState/1 -> MATLAB System1/1
  tIn/1 -> MATLAB System1/2
  speedActual/1 -> RealSim CreatBus/2(speedDesired)
  MATLAB System1/2 -> nMsgSend/1  "nMsgSend"
  rgba/1 -> RealSim CreatBus/3(color)

== system EV6_LUT_FourWheel_EV6Battery77p4kWh_PowerCorrected/Vehicle Under Test1/Environment ==
  Grade : Inport
  Friction : Constant  Value=ones(4,1).*1
  Ground Feedback : Subsystem  Variant=on  VariantControlMode=label  LabelModeActiveChoice=0
  Ground Z Level : Constant  Value=zeros(4,1)
  Subsystem : Subsystem
  Subsystem1 : Subsystem
      mask Display: disp('')
  Env : Outport
  wires:
  Grade/1 -> Subsystem/1(Grade)
  Ground Z Level/1 -> Ground Feedback/2(Ground Z Level)
  Ground Feedback/1(Ground) -> Subsystem1/5(GroundBus)  "Gnd"
  Friction/1 -> Ground Feedback/1(Friction)
  Subsystem1/1(Env) -> Env/1
  Subsystem/1(EnvPrs) -> Subsystem1/1(EnvPrs)
  Subsystem/4(RoadGrade) -> Subsystem1/4(RoadGrade)
  Subsystem/2(EnvTemp) -> Subsystem1/2(EnvTemp)
  Subsystem/3(WindVel) -> Subsystem1/3(WindVel)

== system EV6_LUT_FourWheel_EV6Battery77p4kWh_PowerCorrected/Vehicle Under Test1/Monitor ==
  Monitor : Inport
  Calculate Fuel MPG : Subsystem  Commented=on
  Calculate Powertrain Energy : Subsystem
  Terminator : Terminator
  Terminator3 : Terminator
  wires:
  Calculate Powertrain Energy/1(TransEnrgyOutkWh) -> Terminator3/1  "DiffEnrgyInkWh"
  Monitor/1 -> Calculate Fuel MPG/1(Monitor), Calculate Powertrain Energy/1(Monitor)
  Calculate Fuel MPG/1(FuelEconMPG) -> Terminator/1  "FuelEconMpg"

== system EV6_LUT_FourWheel_EV6Battery77p4kWh_PowerCorrected/Vehicle Under Test1/Performance Calculations ==
  VehSpd : Inport
  BattPwr : Inport  Port=2
  Divide : Product  Inputs=*/
  Divide1 : Product  Inputs=*/
  Divide2 : Product  Inputs=*/
  Integrator : Integrator
  Integrator1 : Integrator
  L/100 Km Calc : Product  Inputs=/*
  Product : Product
  Rate Transition3 : RateTransition  Deterministic=off
  Saturation : Saturate  UpperLimit=Inf  LowerLimit=0.001
  Saturation1 : Saturate  UpperLimit=Inf  LowerLimit=1e-3
  Sqrt : Sqrt
  US EPA kwh/USgal equivalent : Constant  Value=33.7
  US MPG Calc : Product  Inputs=*/
  m to 100Km : Gain  Gain=1/1000/100
  m to mile : Gain  Gain=0.000621371
  m^3 per gal : Gain  Gain=0.00378541
  m^3 to L : Gain  Gain=1000
  m^3 to US Gal : Gain  Gain=264.172
  s per h : Constant  Value=3600
  w per kw : Constant  Value=1000
  US MPG : Outport  VectorParamsAs1DForOutWhenUnconnected=off
  L/100Km : Outport  Port=2  VectorParamsAs1DForOutWhenUnconnected=off
  wires:
  m^3 to US Gal/1 -> Saturation1/1
  m^3 to L/1 -> L/100 Km Calc/2
  Integrator/1 -> m to mile/1, m to 100Km/1
  m to mile/1 -> US MPG Calc/1
  Integrator1/1 -> m^3 to US Gal/1, m^3 to L/1
  Saturation/1 -> L/100 Km Calc/1
  m to 100Km/1 -> Saturation/1
  L/100 Km Calc/1 -> L/100Km/1  "L/100Km"
  US MPG Calc/1 -> Rate Transition3/1
  Saturation1/1 -> US MPG Calc/2
  Rate Transition3/1 -> US MPG/1  "US MPG"
  w per kw/1 -> Divide/2
  Divide/1 -> Divide2/1
  Divide2/1 -> Divide1/1
  s per h/1 -> Divide1/2
  Divide1/1 -> m^3 per gal/1
  m^3 per gal/1 -> Integrator1/1
  US EPA kwh/USgal equivalent/1 -> Divide2/2
  BattPwr/1 -> Divide/1
  Sqrt/1 -> Integrator/1
  Product/1 -> Sqrt/1
  VehSpd/1 -> Product/2, Product/1

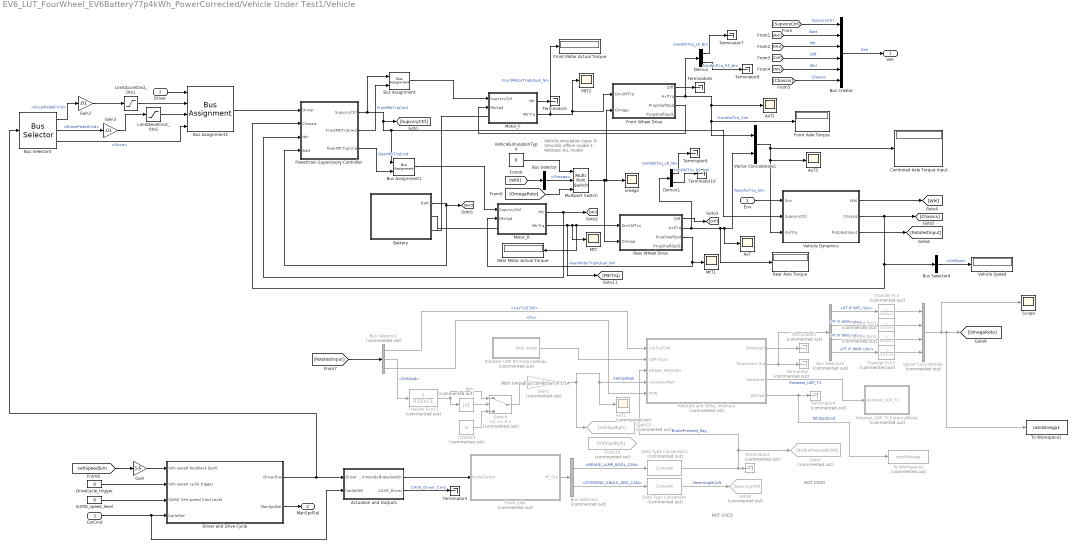
== system EV6_LUT_FourWheel_EV6Battery77p4kWh_PowerCorrected/Vehicle Under Test1/Vehicle ==
  note: NOT USED
  note: Vehicle simulation type:
      | 0- Simulink offline model
      | 1- Rototest HIL model
  note: NOT USED
  note: With tire radius correction of 1.14
  Env : Inport
  Driver : Inport  Port=2
  CarCmd : Inport  Port=3
  Abs : Abs  Commented=on  SaturateOnIntegerOverflow=off
  Actuation and Outputs : Subsystem
  AxT : Scope
  AxT1 : Scope
  AxT2 : Scope  Commented=on
  AxT3 : Scope
  Battery : Subsystem
  Bus Assignment : BusAssignment  AssignedSignals=MtrTrqCmd
  Bus Assignment1 : BusAssignment  AssignedSignals=MtrTrqCmd
  Bus Assignment2 : BusAssignment  AssignedSignals=AccelCmd,DecelCmd,GearCmd
  Bus Creator : BusCreator  Inputs=6
  Bus Selector : BusSelector  OutputSignals=Omega
  Bus Selector1 : BusSelector  Commented=on  OutputSignals=BRAKE_LAMP_BOOL_CAN,STEERING_ANGLE_DEG_CAN
  Bus Selector2 : BusSelector  Commented=on  OutputSignals=CarTrqT2W,VehSpd,Fx
  Bus Selector3 : BusSelector  Commented=on  OutputSignals=PT IF WFL rotv,PT IF WFR rotv,PT IF WRL rotv,PT IF WRR rotv
  Bus Selector4 : BusSelector  OutputSignals=VehSpd
  Bus Selector5 : BusSelector  OutputSignals=AccelPedalCmd,BrakePedalCmd,Drive
  Combined Axle Torque Input : Display
  Constant : Constant  Commented=on  Value=0  SampleTime=-1
  Data Type Conversion : DataTypeConversion  Commented=on  SaturateOnIntegerOverflow=off  RndMeth=Floor
  Data Type Conversion1 : DataTypeConversion  Commented=on  SaturateOnIntegerOverflow=off  RndMeth=Floor
  Demux : Demux  Outputs=2
  Demux1 : Demux  Outputs=2
  DriveCycle_trigger : Constant  Value=0
  Driver and Drive Cycle : Subsystem  TreatAsAtomicUnit=on
  From CAN : Subsystem  Commented=on
  From10 : From  Commented=on  GotoTag=VehSpdKph
  Front Axle Torque : Display
  Front Motor Actual Torque : Display
  Front Wheel Drive : Subsystem  Variant=on  VariantControlMode=label  VariantControl=1  LabelModeActiveChoice=Choice
  Gain : Gain  Gain=3.6
  Gain1 : Gain  Commented=on  Gain=3.6*1.1414
  Gain2 : Gain  Gain=.01
  Gain3 : Gain  Gain=.01
  Goto10 : Goto  Commented=on  GotoTag=VehSpdKph
  Goto7 : Goto  Commented=on  GotoTag=BrakePressedCAN
  Goto8 : Goto  Commented=on  GotoTag=SteeringCAN
  LimitAccelCmd_0to1 : Saturate  UpperLimit=1  LowerLimit=0
  LimitDecelCmd_0to1 : Saturate  UpperLimit=1  LowerLimit=0
  Motor_F : Subsystem
  Motor_R : Subsystem
  MtT : Scope
  MtT1 : Scope
  MtT2 : Scope
  Multiport Switch : MultiPortSwitch  DataPortOrder=Zero-based contiguous  Inputs=2  zeroidx=on  SaturateOnIntegerOverflow=off  InputSameDT=off
  "Powertrain Supervisory Controller " : Subsystem  AncestorBlock=LibPtSupervisoryCtrl/Powertrain Supervisory Controller
  Rear Axle Torque : Display
  Rear Motor Actual Torque : Display
  Rear Wheel Drive : Subsystem  Variant=on  VariantControlMode=label  VariantControl=1  LabelModeActiveChoice=Choice
  "Rototest UDP RX ExternalMode  " : Subsystem  Commented=on
  "Rototest UDP TX ExternalMode  " : Subsystem  Commented=on
  Rototest and ORNL Interface : Subsystem  Commented=on
  SUMO_speed_level : Constant  Value=0
  Scope : Scope
  Switch : Switch  Commented=on  Threshold=0.1  SaturateOnIntegerOverflow=off  InputSameDT=off
  Terminator{,1..2,4} (4 alike) : Terminator  Commented=on
  Terminator{3,5..10} (7 alike) : Terminator
  To Workspace1 : ToWorkspace  VariableName=rotoOmega1  SampleTime=-1
      settings: Save2DSignal=2-D array (concatenate along first dimension)
  To Workspace2 : ToWorkspace  Commented=on  VariableName=rotoOmega  SampleTime=-1
      settings: Save2DSignal=2-D array (concatenate along first dimension)
  Transfer Fcn{,1..3} (4 alike) : TransferFcn  Commented=on  Denominator=[0.01 1]
  Transfer Fcn12 : TransferFcn  Commented=on  Denominator=[0.02 1]
  Vector Concatenate : Concatenate  Commented=on  NumInputs=4
  Vector Concatenate1 : Concatenate
  Vehicle Dynamics : Subsystem  Variant=on  VariantControlMode=label  LabelModeActiveChoice=Veh14DOF  mask{VehDynSel=Vehicle 14DOF}
      mask prompts: VehDynSel "Select the driver"
      mask init:
      | choice = get_param(gcb,'VehDynSel');
      | curBlk = gcb;
      | oldVariant = get_param(gcb,'LabelModeActiveChoice');
      | switch choice
      |     case 'Vehicle Longitudinal'
      |         set_param(curBlk, 'LabelModeActiveChoice', 'VehLong');
      | %     case 'Vehicle 3DOF'   
      | %         set_param(curBlk, 'LabelModeActiveChoice', 'Veh3DOF');
      |     case 'Vehicle 7DOF'   
      |         set_param(curBlk, 'LabelModeActiveChoice', 'Veh7DOF');
      |     case 'Vehicle 14DOF'   
      |         set_param(curBlk, 'LabelModeActiveChoice', 'Veh14DOF');
      | end
      mask TypeOptions VehDynSel: Vehicle Longitudinal | Vehicle 7DOF | Vehicle 14DOF
  Vehicle Speed : Display
  VehicleSimulationType : Constant  Value=0
  omega : Scope
  Veh : Outport
  ManSpdSel : Outport  Port=2
  wires:
  [vehSpeedSim] -> Gain/1
  SUMO_speed_level/1 -> Driver and Drive Cycle/3(SUMO Veh speed Cmd Level)
  Driver and Drive Cycle/2(ManSpdSel) -> ManSpdSel/1
  CarCmd/1 -> Driver and Drive Cycle/4(CarlaRef), Actuation and Outputs/2(CarlaGBS)
  Transfer Fcn12/1 -> Abs/1, Switch/1
  Transfer Fcn3/1 -> Vector Concatenate/4
  Transfer Fcn2/1 -> Vector Concatenate/3
  Transfer Fcn1/1 -> Vector Concatenate/2
  Transfer Fcn/1 -> Vector Concatenate/1
  Abs/1 -> Switch/2
  Switch/1 -> Gain1/1
  Constant/1 -> Switch/3
  Multiport Switch/1 -> Front Wheel Drive/2(Omega), omega/1, Rear Wheel Drive/2(Omega)
  DriveCycle_trigger/1 -> Driver and Drive Cycle/2(Veh speed cycle trigger)
  Gain/1 -> Driver and Drive Cycle/1(Veh speed feedback [kph])
  Gain1/1 -> Goto10/1, Rototest and ORNL Interface/4(vehSpeedKph), AxT2/1  "VehSpdKph"
  [OmegaRoto] -> Multiport Switch/3
  Vector Concatenate/1 -> [OmegaRoto], To Workspace1/1, Scope/1
  Bus Selector3/4 -> Transfer Fcn3/1  "<PT IF WRR rotv>"
  Bus Selector3/3 -> Transfer Fcn2/1  "<PT IF WRL rotv>"
  Bus Selector3/2 -> Transfer Fcn1/1  "<PT IF WFR rotv>"
  Bus Selector3/1 -> Transfer Fcn/1  "<PT IF WFL rotv>"
  Bus Selector/1 -> Multiport Switch/2  "<Omega>"
  Bus Selector2/1 -> Rototest and ORNL Interface/1(CarTrqT2W)  "<CarTrqT2W>"
  Bus Selector2/2 -> Transfer Fcn12/1  "<VehSpd>"
  Bus Selector2/3 -> Rototest and ORNL Interface/5(FXIN)  "<Fx>"
  [RototestInput] -> Bus Selector2/1
  Rototest and ORNL Interface/1(BrakeUpd) -> Terminator1/1
  Rototest and ORNL Interface/3(DataSend) -> "Rototest UDP TX ExternalMode  "/1(Rototest_UDP_TX)  "Rototest_UDP_TX"
  Actuation and Outputs/2(CAVE_Driver) -> Terminator3/1  "CAVE_Driver_Cmd"
  Actuation and Outputs/1(BrakeSwitch) -> From CAN/1(BrakeSwitch)
  From CAN/1(IO_Out) -> Bus Selector1/1
  Bus Selector1/2 -> Data Type Conversion/1  "<STEERING_ANGLE_DEG_CAN>"
  Data Type Conversion1/1 -> Terminator2/1, Goto7/1, Rototest and ORNL Interface/3(BRAKE_PRESSED)  "BrakePressed_flag"
  "Rototest UDP RX ExternalMode  "/1(Data Vector) -> Rototest and ORNL Interface/2(UDP Input)
  Data Type Conversion/1 -> Goto8/1  "SteerAngleCAN"
  Bus Selector1/1 -> Data Type Conversion1/1  "<BRAKE_LAMP_BOOL_CAN>"
  Driver and Drive Cycle/1(DriverBus) -> Bus Selector5/1, Actuation and Outputs/1(Driver Commands)
  VehicleSimulationType/1 -> Multiport Switch/1
  Vehicle Dynamics/3(RototestInput) -> [RototestInput]
  Rototest and ORNL Interface/4(WhlSpd) -> Terminator4/1, To Workspace2/1  "WhlSpdCmd"
  Rototest and ORNL Interface/2(Powertrain Out) -> Terminator/1, Bus Selector3/1
  Rear Wheel Drive/2(AxlTrq) -> Demux1/1, Vector Concatenate1/2, AxT/1, Rear Axle Torque/1  "RearAxlTrq_Sim"
  Motor_R/2(MtrTrq) -> Rear Motor Actual Torque/1, Rear Wheel Drive/1(DrvShfTrq), MtT/1, [MtrTrq]  "RearMotorTrqActual_Nm"
  Rear Wheel Drive/3(PropShaftSpd) -> Motor_R/2(MtrSpd), MtT1/1
  Rear Wheel Drive/1(Diff) -> [Diff]
  [Diff] -> Bus Creator/4  "Diff"
  [Whl] -> Bus Selector/1
  Vehicle Dynamics/1(Whl) -> [Whl]
  Vehicle Dynamics/2(Chassis) -> [Chassis], "Powertrain Supervisory Controller "/2(Chassis), Bus Selector4/1
  Env/1 -> Vehicle Dynamics/1(Env)
  Motor_R/1(Mtr) -> [Mtr], "Powertrain Supervisory Controller "/3(Mtr)
  Battery/1(Batt) -> "Powertrain Supervisory Controller "/4(Batt), [Batt]
  [Chassis] -> Bus Creator/6  "Chassis"
  [Whl] -> Bus Creator/5  "Whl"
  [Mtr] -> Bus Creator/3  "Mtr"
  [Batt] -> Bus Creator/2  "Batt"
  [SupvsryCtrl] -> Bus Creator/1  "SupvsryCtrl"
  Bus Creator/1 -> Veh/1  "Veh"
  "Powertrain Supervisory Controller "/1(SupvsryCtrl) -> Bus Assignment/1, Bus Assignment1/1, Vehicle Dynamics/2(SupvsryCtrl), [SupvsryCtrl]
  Front Wheel Drive/3(PropShaftSpd) -> Motor_F/2(MtrSpd)
  Motor_F/2(MtrTrq) -> MtT2/1, Front Wheel Drive/1(DrvShfTrq), Front Motor Actual Torque/1  "FrontMotorTrqActual_Nm"
  Motor_F/1(Mtr) -> Terminator5/1
  Front Wheel Drive/1(Diff) -> Terminator6/1
  Front Wheel Drive/2(AxlTrq) -> AxT1/1, Vector Concatenate1/1, Front Axle Torque/1, Demux/1  "FrontAxlTrq_Sim"
  Vector Concatenate1/1 -> AxT3/1, Vehicle Dynamics/3(AxlTrq), Combined Axle Torque Input/1
  Bus Selector4/1 -> Vehicle Speed/1  "<VehSpd>"
  "Powertrain Supervisory Controller "/2(FrontMtrTrqCmd) -> Bus Assignment/2  "FrontMtrTrqCmd"
  Bus Assignment/1 -> Motor_F/1(SupvsryCtrl)
  "Powertrain Supervisory Controller "/3(RearMtrTrqCmd) -> Bus Assignment1/2  "RearMtrTrqCmd"
  Bus Assignment1/1 -> Motor_R/1(SupvsryCtrl)
  Bus Assignment2/1 -> "Powertrain Supervisory Controller "/1(Driver)
  Driver/1 -> Bus Assignment2/1
  Bus Selector5/3 -> Bus Assignment2/4  "<Drive>"
  Bus Selector5/2 -> Gain3/1  "<BrakePedalCmd>"
  Bus Selector5/1 -> Gain2/1  "<AccelPedalCmd>"
  Gain3/1 -> LimitDecelCmd_0to1/1
  Gain2/1 -> LimitAccelCmd_0to1/1
  LimitAccelCmd_0to1/1 -> Bus Assignment2/2
  LimitDecelCmd_0to1/1 -> Bus Assignment2/3
  Demux/1 -> Terminator7/1  "SimWhlTrq_LF_Nm"
  Demux/2 -> Terminator8/1  "SimWhlTrq_RF_Nm"
  Demux1/2 -> Terminator10/1  "SimWhlTrq_RR_Nm"
  Demux1/1 -> Terminator9/1  "SimWhlTrq_LR_Nm"
  connections:
  Battery/RConn1 -- Motor_R/LConn1
  Battery/RConn2 -- Motor_F/LConn1
